simulink model "ASM_Traffic_MultiCore"  (R2026a)
settings: Solver=ode1  StartTime=SIM.tstart.v  StopTime=SIM.tend.v  FixedStep=SIM.StepSize.v
PostLoadFcn:
  | if any(exist('dsrtsu_mdlpostloadfcn', 'file') ~= 0), dsrtsu_mdlpostloadfcn('Execute', bdroot); end
  | try, asm_mdl_postloadfcn(bdroot, 'UpdateModel', 3600); catch, disp(lasterr); end,
InitFcn:
  | , if any(exist('rtifpga_mdlclblib', 'file') ~= 0), rtifpga_mdlclblib('Init', bdroot); end,
  | , if any(exist('dsmpb_private', 'file') ~= 0), dsmpb_private('dsmpb_mdlclblib', 'Init', bdroot); end,
model workspace (MAT data in the model file):
  asmReferencePath = [0 0.01 0.02 0.03 0.04 0.05 0.06 0.07 0.08 0.09 0.1 0.11 ... (350007 elements, 50001x7)]
  roadBounds : Simulink.Parameter (value not decoded)
  safetyAxes : Simulink.Parameter (value not decoded)
undefined symbols (not defined in the file): _to_, a0b2, ASM_BrakeHydraulics_DemoSystems, ASM_VehicleDynamics_DemoSystems, b98103fe8ad365046cd0, BrakeCircuit, controllerConfig, CPT, Crankshaft, DiscIntNeverNeededParam, dsmsi, FinalDriveAssembly, MDL, ModeSignals, mu, Pos_BrakePedal_Maneuver, rad, RefSignals, roadFamilyData, roadFamilyId, s_to_rpm, SIM, SoftECU, Suspension, Tire, Transmission
libraries: ASM_Traffic_lib x135, simulink x98, ASM_Utils_lib x77, ASM_VehicleDynamics_lib x70, ASM_Environment_lib x22, dsmpblib x20, dsmsilib x15, MDLD_Utils_lib x10, ASM_BrakeHydraulics_lib x3, sl_discontinuities x2
(part 27 of 65)

== system ASM_Traffic_MultiCore/Environment/Interface_Out/Plant_ModelSignals/Sw_TipShift_Maneuver[-1Down|0Off|1Up]_ ==
  In1 : Inport
  DummyGain : Gain  SaturateOnIntegerOverflow=on  OutDataTypeStr=Inherit: Same as input  ParamDataTypeStr=Inherit: Same as input
  Out1 : Outport  VectorParamsAs1DForOutWhenUnconnected=off
  wires:
  In1/1 -> DummyGain/1
  DummyGain/1 -> Out1/1

== system ASM_Traffic_MultiCore/Environment/Interface_Out/Plant_ModelSignals/Sw_Tire_Parameter_Set_CP[:][1|2|3|4]_ ==
  In1 : Inport
  Gain : Gain  SaturateOnIntegerOverflow=on  OutDataTypeStr=Inherit: Same as input  ParamDataTypeStr=Inherit: Same as input
  Out1 : Outport  VectorParamsAs1DForOutWhenUnconnected=off
  wires:
  In1/1 -> Gain/1
  Gain/1 -> Out1/1

== system ASM_Traffic_MultiCore/Environment/Interface_Out/Plant_ModelSignals/T_Ambient[degC]_ ==
  In1 : Inport
  Gain : Gain  SaturateOnIntegerOverflow=on  OutDataTypeStr=Inherit: Same as input  ParamDataTypeStr=Inherit: Same as input
  Out1 : Outport  VectorParamsAs1DForOutWhenUnconnected=off
  wires:
  In1/1 -> Gain/1
  Gain/1 -> Out1/1

== system ASM_Traffic_MultiCore/Environment/Interface_Out/Plant_ModelSignals/Trq_Driver_External[Nm]_ ==
  In1 : Inport
  Gain : Gain  SaturateOnIntegerOverflow=on  OutDataTypeStr=Inherit: Same as input  ParamDataTypeStr=Inherit: Same as input
  Out1 : Outport  VectorParamsAs1DForOutWhenUnconnected=off
  wires:
  In1/1 -> Gain/1
  Gain/1 -> Out1/1

== system ASM_Traffic_MultiCore/Environment/Interface_Out/Plant_ModelSignals/UnitVec_z_CP[:][x;y;z]_ ==
  In1 : Inport
  Gain : Gain  SaturateOnIntegerOverflow=on  OutDataTypeStr=Inherit: Same as input  ParamDataTypeStr=Inherit: Same as input
  Out1 : Outport  VectorParamsAs1DForOutWhenUnconnected=off
  wires:
  In1/1 -> Gain/1
  Gain/1 -> Out1/1

== system ASM_Traffic_MultiCore/Environment/Interface_Out/Plant_ModelSignals/Width_Deadzone_LatCtrl[m]_ ==
  In1 : Inport
  Gain : Gain  SaturateOnIntegerOverflow=on  OutDataTypeStr=Inherit: Same as input  ParamDataTypeStr=Inherit: Same as input
  Out1 : Outport  VectorParamsAs1DForOutWhenUnconnected=off
  wires:
  In1/1 -> Gain/1
  Gain/1 -> Out1/1

== system ASM_Traffic_MultiCore/Environment/Interface_Out/Plant_ModelSignals/Width_Fellows[m]_ ==
  In1 : Inport
  Gain : Gain  SaturateOnIntegerOverflow=on  OutDataTypeStr=Inherit: Same as input  ParamDataTypeStr=Inherit: Same as input
  Out1 : Outport  VectorParamsAs1DForOutWhenUnconnected=off
  wires:
  In1/1 -> Gain/1
  Gain/1 -> Out1/1

== system ASM_Traffic_MultiCore/Environment/Interface_Out/Plant_ModelSignals/a_x_Max[m|s2]_ ==
  In1 : Inport
  DummyGain : Gain  SaturateOnIntegerOverflow=on  OutDataTypeStr=Inherit: Same as input  ParamDataTypeStr=Inherit: Same as input
  Out1 : Outport  VectorParamsAs1DForOutWhenUnconnected=off
  wires:
  DummyGain/1 -> Out1/1
  In1/1 -> DummyGain/1

== system ASM_Traffic_MultiCore/Environment/Interface_Out/Plant_ModelSignals/a_x_Min[m|s2]_ ==
  In1 : Inport
  DummyGain : Gain  SaturateOnIntegerOverflow=on  OutDataTypeStr=Inherit: Same as input  ParamDataTypeStr=Inherit: Same as input
  Out1 : Outport  VectorParamsAs1DForOutWhenUnconnected=off
  wires:
  In1/1 -> DummyGain/1
  DummyGain/1 -> Out1/1

== system ASM_Traffic_MultiCore/Environment/Interface_Out/Plant_ModelSignals/a_x_Vehicle_Ref_TrafficDriver[m|s2]_ ==
  In1 : Inport
  Gain : Gain  SaturateOnIntegerOverflow=on  OutDataTypeStr=Inherit: Same as input  ParamDataTypeStr=Inherit: Same as input
  Out1 : Outport  VectorParamsAs1DForOutWhenUnconnected=off
  wires:
  Gain/1 -> Out1/1
  In1/1 -> Gain/1

== system ASM_Traffic_MultiCore/Environment/Interface_Out/Plant_ModelSignals/a_y_Max[m|s2]_ ==
  In1 : Inport
  DummyGain : Gain  SaturateOnIntegerOverflow=on  OutDataTypeStr=Inherit: Same as input  ParamDataTypeStr=Inherit: Same as input
  Out1 : Outport  VectorParamsAs1DForOutWhenUnconnected=off
  wires:
  DummyGain/1 -> Out1/1
  In1/1 -> DummyGain/1

== system ASM_Traffic_MultiCore/Environment/Interface_Out/Plant_ModelSignals/d_Total_Fellows[m]_ ==
  In1 : Inport
  Gain : Gain  SaturateOnIntegerOverflow=on  OutDataTypeStr=Inherit: Same as input  ParamDataTypeStr=Inherit: Same as input
  Out1 : Outport  VectorParamsAs1DForOutWhenUnconnected=off
  wires:
  In1/1 -> Gain/1
  Gain/1 -> Out1/1

== system ASM_Traffic_MultiCore/Environment/Interface_Out/Plant_ModelSignals/d_Vehicle_Road[m]_ ==
  In1 : Inport
  Gain : Gain  SaturateOnIntegerOverflow=on  OutDataTypeStr=Inherit: Same as input  ParamDataTypeStr=Inherit: Same as input
  Out1 : Outport  VectorParamsAs1DForOutWhenUnconnected=off
  wires:
  In1/1 -> Gain/1
  Gain/1 -> Out1/1

== system ASM_Traffic_MultiCore/Environment/Interface_Out/Plant_ModelSignals/n_Engine_Set[rpm]_ ==
  In1 : Inport
  DummyGain : Gain  SaturateOnIntegerOverflow=on  OutDataTypeStr=Inherit: Same as input  ParamDataTypeStr=Inherit: Same as input
  Out1 : Outport  VectorParamsAs1DForOutWhenUnconnected=off
  wires:
  In1/1 -> DummyGain/1
  DummyGain/1 -> Out1/1

== system ASM_Traffic_MultiCore/Environment/Interface_Out/Plant_ModelSignals/p_Ambient[Pa]_ ==
  In1 : Inport
  Gain : Gain  SaturateOnIntegerOverflow=on  OutDataTypeStr=Inherit: Same as input  ParamDataTypeStr=Inherit: Same as input
  Out1 : Outport  VectorParamsAs1DForOutWhenUnconnected=off
  wires:
  In1/1 -> Gain/1
  Gain/1 -> Out1/1

== system ASM_Traffic_MultiCore/Environment/Interface_Out/Plant_ModelSignals/q_dt_Vehicle_Init[6x1]_ ==
  In1 : Inport
  Gain : Gain  SaturateOnIntegerOverflow=on  OutDataTypeStr=Inherit: Same as input  ParamDataTypeStr=Inherit: Same as input
  Out1 : Outport  VectorParamsAs1DForOutWhenUnconnected=off
  wires:
  In1/1 -> Gain/1
  Gain/1 -> Out1/1

== system ASM_Traffic_MultiCore/Environment/Interface_Out/Plant_ModelSignals/s_Fellows_Ref[m]_ ==
  In1 : Inport
  Gain : Gain  SaturateOnIntegerOverflow=on  OutDataTypeStr=Inherit: Same as input  ParamDataTypeStr=Inherit: Same as input
  Out1 : Outport  VectorParamsAs1DForOutWhenUnconnected=off
  wires:
  In1/1 -> Gain/1
  Gain/1 -> Out1/1

== system ASM_Traffic_MultiCore/Environment/Interface_Out/Plant_ModelSignals/s_Total_Vehicle_Road[m]_ ==
  In1 : Inport
  Gain : Gain  SaturateOnIntegerOverflow=on  OutDataTypeStr=Inherit: Same as input  ParamDataTypeStr=Inherit: Same as input
  Out1 : Outport  VectorParamsAs1DForOutWhenUnconnected=off
  wires:
  Gain/1 -> Out1/1
  In1/1 -> Gain/1

== system ASM_Traffic_MultiCore/Environment/Interface_Out/Plant_ModelSignals/s_Vehicle_Init[m]_ ==
  In1 : Inport
  Gain : Gain  SaturateOnIntegerOverflow=on  OutDataTypeStr=Inherit: Same as input  ParamDataTypeStr=Inherit: Same as input
  Out1 : Outport  VectorParamsAs1DForOutWhenUnconnected=off
  wires:
  Gain/1 -> Out1/1
  In1/1 -> Gain/1

== system ASM_Traffic_MultiCore/Environment/Interface_Out/Plant_ModelSignals/s_Vehicle_Road[m]_ ==
  In1 : Inport
  Gain : Gain  SaturateOnIntegerOverflow=on  OutDataTypeStr=Inherit: Same as input  ParamDataTypeStr=Inherit: Same as input
  Out1 : Outport  VectorParamsAs1DForOutWhenUnconnected=off
  wires:
  In1/1 -> Gain/1
  Gain/1 -> Out1/1

== system ASM_Traffic_MultiCore/Environment/Interface_Out/Plant_ModelSignals/v_Rel_Fellows[m|s]_ ==
  In1 : Inport
  Gain : Gain  SaturateOnIntegerOverflow=on  OutDataTypeStr=Inherit: Same as input  ParamDataTypeStr=Inherit: Same as input
  Out1 : Outport  VectorParamsAs1DForOutWhenUnconnected=off
  wires:
  In1/1 -> Gain/1
  Gain/1 -> Out1/1

== system ASM_Traffic_MultiCore/Environment/Interface_Out/Plant_ModelSignals/v_Vehicle_Preview_Ref_Maneuver[m|s]_ ==
  In1 : Inport
  DummyGain : Gain  SaturateOnIntegerOverflow=on  OutDataTypeStr=Inherit: Same as input  ParamDataTypeStr=Inherit: Same as input
  Out1 : Outport  VectorParamsAs1DForOutWhenUnconnected=off
  wires:
  In1/1 -> DummyGain/1
  DummyGain/1 -> Out1/1

== system ASM_Traffic_MultiCore/Environment/Interface_Out/Plant_ModelSignals/v_Vehicle_Ref_Maneuver[km|h]_ ==
  In1 : Inport
  DummyGain : Gain  SaturateOnIntegerOverflow=on  OutDataTypeStr=Inherit: Same as input  ParamDataTypeStr=Inherit: Same as input
  Out1 : Outport  VectorParamsAs1DForOutWhenUnconnected=off
  wires:
  DummyGain/1 -> Out1/1
  In1/1 -> DummyGain/1

== system ASM_Traffic_MultiCore/Environment/Interface_Out/Plant_ModelSignals/v_Wind_Coor_Sys_E[x;y;z][m|s]_ ==
  In1 : Inport
  Gain : Gain  SaturateOnIntegerOverflow=on  OutDataTypeStr=Inherit: Same as input  ParamDataTypeStr=Inherit: Same as input
  Out1 : Outport  VectorParamsAs1DForOutWhenUnconnected=off
  wires:
  In1/1 -> Gain/1
  Gain/1 -> Out1/1

== system ASM_Traffic_MultiCore/Environment/Interface_Out/Plant_ModelSignals/x_Preview_DriverCurv[m]_ ==
  In1 : Inport
  Gain : Gain  SaturateOnIntegerOverflow=on  OutDataTypeStr=Inherit: Same as input  ParamDataTypeStr=Inherit: Same as input
  Out1 : Outport  VectorParamsAs1DForOutWhenUnconnected=off
  wires:
  In1/1 -> Gain/1
  Gain/1 -> Out1/1

== system ASM_Traffic_MultiCore/Environment/Interface_Out/Plant_ModelSignals/y_Preview_DriverCurv[m]_ ==
  In1 : Inport
  Gain : Gain  SaturateOnIntegerOverflow=on  OutDataTypeStr=Inherit: Same as input  ParamDataTypeStr=Inherit: Same as input
  Out1 : Outport  VectorParamsAs1DForOutWhenUnconnected=off
  wires:
  Gain/1 -> Out1/1
  In1/1 -> Gain/1

== system ASM_Traffic_MultiCore/Environment/Maneuver/PlantModel/ASMSignalCollector ==
  UserInterface : Inport
  VehicleInitStates : Inport  Port=2
  ModeSignals : Inport  Port=3
  RefSignals : Inport  Port=4
  Bus Creator : BusCreator  Inputs=7
  Bus Selector8 : BusSelector  OutputSignals=ManualControl.Testbench,ManualControl.ParkingBrake,ManualControl.StartButton,ManualControl.AutomaticTransmission.Sw_TipShift[-1Down|0Off|1Up]
  Replace_ModeSignals : BusAssignment  AssignedSignals=ModeSignals,RefSignals
  Maneuver_Signals : Outport  VectorParamsAs1DForOutWhenUnconnected=off
  wires:
  VehicleInitStates/1 -> Bus Creator/3
  Bus Selector8/1 -> Bus Creator/4  "<Testbench>"
  Bus Creator/1 -> Maneuver_Signals/1  "Maneuver"
  [ASMBUS_Environment_Mnvr_UserSignalsCustomized] -> Bus Creator/2
  [ASMBUS_Environment_ManeuverScheduler] -> Replace_ModeSignals/1
  Bus Selector8/2 -> Bus Creator/5  "<ParkingBrake>"
  Bus Selector8/3 -> Bus Creator/6  "<StartButton>"
  Bus Selector8/4 -> Bus Creator/7  "<Sw_TipShift[-1Down|0Off|1Up]>"
  ModeSignals/1 -> Replace_ModeSignals/2
  RefSignals/1 -> Replace_ModeSignals/3
  Replace_ModeSignals/1 -> Bus Creator/1  "ManeuverScheduler"
  UserInterface/1 -> Bus Selector8/1

== system ASM_Traffic_MultiCore/Environment/Maneuver/PlantModel/Customize_UserSignals ==
  UserSignals_In : Inport
  Bus Creator : BusCreator  Inputs=14
  Bus Selector1 : BusSelector  OutputSignals=User1[],User2[],User3[],User4[],User5[],User6[],User7[],User8[],User9[],User10[],User11[],User12[],User13[],User14[]
  CustomizedUserSignals : Subsystem
  ASMSignalBus : Outport  VectorParamsAs1DForOutWhenUnconnected=off
  UserSignals_Customized : Outport  Port=2  VectorParamsAs1DForOutWhenUnconnected=off
  wires:
  CustomizedUserSignals/8(Mnv_DataStream_8[]) -> Bus Creator/8
  CustomizedUserSignals/7(Mnv_DataStream_7[]) -> Bus Creator/7
  CustomizedUserSignals/6(Mnv_DataStream_6[]) -> Bus Creator/6
  CustomizedUserSignals/5(Mnv_DataStream_5[]) -> Bus Creator/5
  Bus Selector1/8 -> CustomizedUserSignals/8(User8[])  "<User8[]>"
  Bus Selector1/7 -> CustomizedUserSignals/7(User7[])  "<User7[]>"
  Bus Selector1/6 -> CustomizedUserSignals/6(User6[])  "<User6[]>"
  Bus Selector1/5 -> CustomizedUserSignals/5(User5[])  "<User5[]>"
  Bus Selector1/4 -> CustomizedUserSignals/4(User4[])  "<User4[]>"
  Bus Selector1/3 -> CustomizedUserSignals/3(User3[])  "<User3[]>"
  CustomizedUserSignals/3(ASM_Vehicle_TurnLights[]) -> Bus Creator/3
  CustomizedUserSignals/4(ECU_Commands[]) -> Bus Creator/4
  UserSignals_In/1 -> Bus Selector1/1
  Bus Creator/1 -> ASMSignalBus/1, UserSignals_Customized/1  "UserSignals_Customized"
  Bus Selector1/1 -> CustomizedUserSignals/1(User1[])  "<User1[]>"
  Bus Selector1/2 -> CustomizedUserSignals/2(User2[])  "<User2[]>"
  CustomizedUserSignals/1(ExternalSegmentEnd_Mode[]) -> Bus Creator/1
  CustomizedUserSignals/2(ExternalSegmentEnd_Value[]) -> Bus Creator/2
  Bus Selector1/9 -> CustomizedUserSignals/9(User9[])  "<User9[]>"
  Bus Selector1/10 -> CustomizedUserSignals/10(User10[])  "<User10[]>"
  Bus Selector1/11 -> CustomizedUserSignals/11(User11[])  "<User11[]>"
  Bus Selector1/12 -> CustomizedUserSignals/12(User12[])  "<User12[]>"
  Bus Selector1/13 -> CustomizedUserSignals/13(User13[])  "<User13[]>"
  Bus Selector1/14 -> CustomizedUserSignals/14(User14[])  "<User14[]>"
  CustomizedUserSignals/9(Mnv_DoorFL[]) -> Bus Creator/9
  CustomizedUserSignals/10(Mnv_DoorFR[]) -> Bus Creator/10
  CustomizedUserSignals/11(Mnv_DoorRL[]) -> Bus Creator/11
  CustomizedUserSignals/12(Mnv_DoorRR[]) -> Bus Creator/12
  CustomizedUserSignals/13(Mnv_Hood[]) -> Bus Creator/13
  CustomizedUserSignals/14(Mnv_Trunk[]) -> Bus Creator/14

== system ASM_Traffic_MultiCore/Environment/Maneuver/PlantModel/ExternalSegmentEnd ==
  In : Inport
  UserSignals_Customized : Inport  Port=2
  AvoidAlgLoop{1..9} (9 alike) : UnitDelay  SampleTime=-1
  Bus Selector : BusSelector  OutputSignals=ExternalSegmentEnd_Mode[],ExternalSegmentEnd_Value[]
  Bus Selector1 : BusSelector  OutputSignals=Plant.Traffic_Signals_toEnvironment.UserSignals_Customized.ManeuverSegmentEndTrigger[0|1]
  Bus Selector2 : BusSelector  OutputSignals=Plant.Road_ASMVeh.s_Veh_Road[m]
  Bus Selector3 : BusSelector  OutputSignals=Road,Interface_In,Sensors,Traffic
  Bus Selector4 : BusSelector  OutputSignals=ExternalModel.RollRate_Vehicle_CoG[deg|s]
  Bus Selector5 : BusSelector  OutputSignals=Plant.Object_Sensor_3D.Sensor_1_Front_Long,Plant.Object_Sensor_3D.Sensor_3_Rear
  Bus Selector6 : BusSelector  OutputSignals=ExternalModel.AEB[0|1],ExternalModel.FCW[0|1]
  Bus Selector7 : BusSelector  OutputSignals=SensorOutput.Dist_Object[m]
  Bus Selector8 : BusSelector  OutputSignals=SensorOutput.Dist_Object[m]
  Const_External_SegmentEnd_10[0|1] : Constant  Value=0
  Const_External_SegmentEnd_11_25 : Constant  Value=zeros(15,1)
  Const_External_SegmentEnd_5[0|1] : Constant  Value=0
  Const_External_SegmentEnd_6[0|1] : Constant  Value=0
  Const_External_SegmentEnd_7[0|1] : Constant  Value=0
  Const_External_SegmentEnd_8[0|1] : Constant  Value=0
  Const_External_SegmentEnd_9[0|1] : Constant  Value=0
  Dist_Front_Min : Subsystem
  Dist_Rear_Min : Subsystem
  Mux : Mux  Inputs=[1 1 1 1 1 1 1 1 1 1 15]
  SegmentEndTrigger : Subsystem
  External_SegmentEnd[0|1] : Outport  VectorParamsAs1DForOutWhenUnconnected=off
  wires:
  Bus Selector7/1 -> Dist_Front_Min/1(Dist_Front[m])  "<Dist_Object[m]>"
  AvoidAlgLoop9/1 -> Mux/4
  AvoidAlgLoop8/1 -> Mux/3
  Bus Selector6/2 -> AvoidAlgLoop9/1  "<FCW[0|1]>"
  Bus Selector6/1 -> AvoidAlgLoop8/1  "<AEB[0|1]>"
  Const_External_SegmentEnd_5[0|1]/1 -> Mux/5
  Const_External_SegmentEnd_6[0|1]/1 -> Mux/6
  Const_External_SegmentEnd_7[0|1]/1 -> Mux/7
  Const_External_SegmentEnd_8[0|1]/1 -> Mux/8
  Const_External_SegmentEnd_9[0|1]/1 -> Mux/9
  Const_External_SegmentEnd_10[0|1]/1 -> Mux/10
  Mux/1 -> External_SegmentEnd[0|1]/1
  Bus Selector3/4 -> Bus Selector1/1  "<Traffic>"
  Bus Selector1/1 -> AvoidAlgLoop6/1  "<ManeuverSegmentEndTrigger[0|1]>"
  AvoidAlgLoop6/1 -> Mux/2
  UserSignals_Customized/1 -> Bus Selector/1
  Bus Selector/1 -> AvoidAlgLoop1/1  "<ExternalSegmentEnd_Mode[]>"
  Bus Selector/2 -> AvoidAlgLoop2/1  "<ExternalSegmentEnd_Value[]>"
  Bus Selector3/2 -> Bus Selector6/1, Bus Selector4/1  "<Interface_In>"
  Bus Selector4/1 -> AvoidAlgLoop4/1  "<RollRate_Vehicle_CoG[deg|s]>"
  Bus Selector2/1 -> AvoidAlgLoop3/1  "<s_Veh_Road[m]>"
  AvoidAlgLoop1/1 -> SegmentEndTrigger/1(ExternalSegmentEnd_Mode[])
  AvoidAlgLoop2/1 -> SegmentEndTrigger/2(ExternalSegmentEnd_Value[])
  AvoidAlgLoop3/1 -> SegmentEndTrigger/3(s_Road[m])
  AvoidAlgLoop4/1 -> SegmentEndTrigger/4(RollRate_Vehicle[deg|s])
  Dist_Front_Min/1(Out1) -> AvoidAlgLoop5/1
  Dist_Rear_Min/1(Out1) -> AvoidAlgLoop7/1
  AvoidAlgLoop7/1 -> SegmentEndTrigger/6(Distance_Rear[m])
  AvoidAlgLoop5/1 -> SegmentEndTrigger/5(Distance_Front[m])
  SegmentEndTrigger/1(External_SegmentEnd[0|1]) -> Mux/1
  Const_External_SegmentEnd_11_25/1 -> Mux/11
  In/1 -> Bus Selector3/1
  Bus Selector3/1 -> Bus Selector2/1  "<Road>"
  Bus Selector3/3 -> Bus Selector5/1  "<Sensors>"
  Bus Selector5/1 -> Bus Selector7/1  "<Sensor_1_Front_Long>"
  Bus Selector5/2 -> Bus Selector8/1  "<Sensor_3_Rear>"
  Bus Selector8/1 -> Dist_Rear_Min/1(Dist_Rear[m])  "<Dist_Object[m]>"

== system ASM_Traffic_MultiCore/Environment/Maneuver/PlantModel/ExternalUserData ==
  Angle_SteeringWheel[deg] : Constant  Value=0
  Bus Creator2 : BusCreator  Inputs=10
  Gear[] : Constant  Value=0
  LaneIdx_Ref[] : Constant  Value=0
  Pos_AccPedal[%] : Constant  Value=0
  Pos_BrakePedal[%] : Constant  Value=0
  Pos_ClutchPedal[%] : Constant  Value=100
  "SelectorLever[] " : Constant  Value=0
  Trq_Steering[Nm] : Constant  Value=0
  d_Ref[m] : Constant  Value=0
  v_Vehicle_Ref[m|s] : Constant  Value=0
  External_ReferenceSignals : Outport  VectorParamsAs1DForOutWhenUnconnected=off
  wires:
  "SelectorLever[] "/1 -> Bus Creator2/10  "SelectorLever[]"
  Trq_Steering[Nm]/1 -> Bus Creator2/9  "Trq_Steering[Nm]"
  Angle_SteeringWheel[deg]/1 -> Bus Creator2/5  "Angle_SteeringWheel[deg]"
  Gear[]/1 -> Bus Creator2/4  "Gear[]"
  Pos_ClutchPedal[%]/1 -> Bus Creator2/3  "Pos_ClutchPedal[%]"
  Pos_BrakePedal[%]/1 -> Bus Creator2/2  "Pos_BrakePedal[%]"
  Pos_AccPedal[%]/1 -> Bus Creator2/1  "Pos_AccPedal[%]"
  v_Vehicle_Ref[m|s]/1 -> Bus Creator2/6  "v_Vehicle_Ref[m|s]"
  d_Ref[m]/1 -> Bus Creator2/7  "d_Ref[m]"
  LaneIdx_Ref[]/1 -> Bus Creator2/8  "LaneIdx_Ref[]"
  Bus Creator2/1 -> External_ReferenceSignals/1

== system ASM_Traffic_MultiCore/Environment/Maneuver/PlantModel/InitialVehicleStates ==
  note: Set v_x_Init to zero if Keep_VehiclePosition is enabled or the maneuver state is BRAKE or WAIT.
  note: Use v_x_Init from VehicleInitStates_External if the maneuver state is INIT_MANUAL or MANUAL; else use v_x_Init from the maneuver scheduler.
  UserInterface : Inport
  MdlControl : Inport  Port=2
  InitialVehStates : Inport  Port=3
  Info[] : Inport  Port=4
  Bus Creator1 : BusCreator  Inputs=2
  Bus Selector10 : BusSelector  OutputSignals=Vehicle_Init
  Bus Selector2 : BusSelector  OutputSignals=v_Vehicle_Init[km|h]
  Bus Selector3 : BusSelector  OutputSignals=Keep_VehiclePosition[0|1]
  Bus Selector4 : BusSelector  OutputSignals=Reset_VehicleStates[0|1]
  Bus Selector5 : BusSelector  OutputSignals=ManeuverState[],CurrentSequence[],CurrentSegment[]
  Bus to Vector : BusToVector
  Const_zero_v_x_Init[km|h] : Constant  Value=0  VectorParams1D=off
  DRIVETRAIN_INIT : ASM_Environment_lib/Environment/Maneuver/DRIVETRAIN_INIT  StepSize=SIM.StepSize  ASMProperties=struct('Name','DRIVETRAIN_INIT','Version','1.0','Library','ASM_Environment_lib')  ASMInstanceName=drivetrain_init  ASMInstanceID=1
  Demux : Demux  Outputs=[1 1 1 3]
  Keep_VehiclePosition_enabled : simulink/Logic and Bit Operations/Compare To Constant  relop===  const=1  OutDataTypeStr=uint8  ZeroCross=off
  Mux : Mux  Inputs=3
  Mux1 : Mux  Inputs=[3 3]
  OR : Logic  Operator=OR  Inputs=3  IconShape=distinctive  AllPortsSameDT=off  OutDataTypeStr=boolean
  OR1 : Logic  Operator=OR  IconShape=distinctive  AllPortsSameDT=off  OutDataTypeStr=boolean
  State_BRAKE : simulink/Logic and Bit Operations/Compare To Constant  relop===  const=4  OutDataTypeStr=uint8  ZeroCross=off
  State_INIT_MANUAL : simulink/Logic and Bit Operations/Compare To Constant  relop===  const=6  OutDataTypeStr=uint8  ZeroCross=off
  State_MANUAL : simulink/Logic and Bit Operations/Compare To Constant  relop===  const=7  OutDataTypeStr=uint8  ZeroCross=off
  State_WAIT : simulink/Logic and Bit Operations/Compare To Constant  relop===  const=5  OutDataTypeStr=uint8  ZeroCross=off
  Sw_KeepVehiclePosition_Dependency : Gain
  Sw_ManeuverState_Dependency : Gain
  Switch : Switch  Criteria=u2 ~= 0  SaturateOnIntegerOverflow=off  InputSameDT=off
  Switch1 : Switch  Criteria=u2 ~= 0  SaturateOnIntegerOverflow=off  InputSameDT=off
  Unit Delay : UnitDelay  SampleTime=-1
  UnitConversion : ASM_Utils_lib/UnitConversion/UnitConversion  Selection=km/h_to_m/s
  VehicleInitStates : Outport  VectorParamsAs1DForOutWhenUnconnected=off
  Flag_Init_Drivetrain[0InProgress|1Finished] : Outport  Port=2  VectorParamsAs1DForOutWhenUnconnected=off
  wires:
  Demux/3 -> Mux/3  "vz"
  Demux/2 -> Mux/2  "vy"
  Bus Creator1/1 -> VehicleInitStates/1  "VehicleInitStates"
  Mux/1 -> UnitConversion/1
  Demux/4 -> Mux1/2  "w_Init[x;y;z][rad|s]"
  Unit Delay/1 -> Mux/1  "vx"
  Mux1/1 -> Bus Creator1/1  "q_dt_Vehicle_Init[6x1]"
  Demux/1 -> Switch1/1
  State_BRAKE/1 -> OR/2
  State_WAIT/1 -> OR/3
  Sw_ManeuverState_Dependency/1 -> State_BRAKE/1, State_MANUAL/1, State_INIT_MANUAL/1, State_WAIT/1
  Sw_KeepVehiclePosition_Dependency/1 -> Keep_VehiclePosition_enabled/1
  Keep_VehiclePosition_enabled/1 -> OR/1
  OR/1 -> Switch/2
  Switch1/1 -> Switch/3
  Switch/1 -> Unit Delay/1
  State_INIT_MANUAL/1 -> OR1/1
  State_MANUAL/1 -> OR1/2
  OR1/1 -> Switch1/2
  Bus to Vector/1 -> Demux/1
  UnitConversion/1 -> Mux1/1  "v_Init[x;y;z][m|s]"
  Bus Selector10/1 -> Bus to Vector/1  "<Vehicle_Init>"
  UserInterface/1 -> Bus Selector10/1
  Bus Selector3/1 -> Sw_KeepVehiclePosition_Dependency/1  "<Keep_VehiclePosition[0|1]>"
  MdlControl/1 -> Bus Selector4/1, Bus Selector3/1
  Bus Selector2/1 -> DRIVETRAIN_INIT/1, Switch1/3  "<v_Vehicle_Init[km|h]>"
  InitialVehStates/1 -> Bus Selector2/1
  Const_zero_v_x_Init[km|h]/1 -> Switch/1
  Bus Selector5/3 -> DRIVETRAIN_INIT/4  "<CurrentSegment[]>"
  Bus Selector5/1 -> Sw_ManeuverState_Dependency/1, DRIVETRAIN_INIT/2  "<ManeuverState[]>"
  Bus Selector5/2 -> DRIVETRAIN_INIT/3  "<CurrentSequence[]>"
  Info[]/1 -> Bus Selector5/1
  Bus Selector4/1 -> DRIVETRAIN_INIT/5  "<Reset_VehicleStates[0|1]>"
  DRIVETRAIN_INIT/1 -> Bus Creator1/2  "Enable_v_Init[0|1]"
  DRIVETRAIN_INIT/2 -> Flag_Init_Drivetrain[0InProgress|1Finished]/1

== system ASM_Traffic_MultiCore/Environment/Maneuver/PlantModel/LastValues ==
  In : Inport
  Maneuver_RefSignals : Inport  Port=2
  AvoidAlgLoop_AccPed : UnitDelay  SampleTime=-1
  AvoidAlgLoop_BrakePed : UnitDelay  SampleTime=-1
  AvoidAlgLoop_ClutchPed : UnitDelay  SampleTime=-1
  AvoidAlgLoop_Gear : UnitDelay  SampleTime=-1
  AvoidAlgLoop_Steer{,1..4} (5 alike) : UnitDelay  SampleTime=-1
  Bus Creator3 : BusCreator  Inputs=9
  Bus Selector1 : BusSelector  OutputSignals=ExternalModel.Angle_SteeringWheel_SteeringSystem[deg],ExternalModel.Trq_SteeringWheel_SteeringSystem[Nm]
  Bus Selector2 : BusSelector  OutputSignals=ExternalModel.Pos_AccPedal[%],ExternalModel.Pos_BrakePedal[%],ExternalModel.Pos_ClutchPedal[%],ExternalModel.Gear[],ExternalModel.SelectorLever[-3T|-2P|-1R|0N|1D],ExternalModel.Angle_SteeringWheel[deg]
  Bus Selector3 : BusSelector  OutputSignals=Sw_SteeringMode_Maneuver[1Angle|2Trq]
  Bus Selector4 : BusSelector  OutputSignals=Interface_In,Road
  Bus Selector5 : BusSelector  OutputSignals=Plant.Road_ASMVeh.d_Total_Veh_Road[m],Plant.Road_ASMVeh.LaneIdx_Total_Veh_Road[]
  Multiport Switch : MultiPortSwitch  Inputs=2  SaturateOnIntegerOverflow=off  InputSameDT=off
  LastValues : Outport  VectorParamsAs1DForOutWhenUnconnected=off
  wires:
  Bus Selector5/1 -> AvoidAlgLoop_Steer1/1  "<d_Total_Veh_Road[m]>"
  Bus Selector5/2 -> AvoidAlgLoop_Steer2/1  "<LaneIdx_Total_Veh_Road[]>"
  Bus Creator3/1 -> LastValues/1
  AvoidAlgLoop_Steer2/1 -> Bus Creator3/7  "LaneIdx_Total_Veh_Road_Last[]"
  AvoidAlgLoop_Steer1/1 -> Bus Creator3/6  "d_Total_Veh_Road_Last[m]"
  AvoidAlgLoop_Steer/1 -> Bus Creator3/5  "Angle_SteeringWheel_Last[deg]"
  AvoidAlgLoop_Gear/1 -> Bus Creator3/4  "Gear_Last[]"
  AvoidAlgLoop_ClutchPed/1 -> Bus Creator3/3  "Pos_ClutchPedal_Last[%]"
  AvoidAlgLoop_BrakePed/1 -> Bus Creator3/2  "Pos_BrakePedal_Last[%]"
  AvoidAlgLoop_AccPed/1 -> Bus Creator3/1  "Pos_AccPedal_Last[%]"
  Bus Selector2/1 -> AvoidAlgLoop_AccPed/1  "<Pos_AccPedal[%]>"
  Bus Selector2/2 -> AvoidAlgLoop_BrakePed/1  "<Pos_BrakePedal[%]>"
  Bus Selector2/3 -> AvoidAlgLoop_ClutchPed/1  "<Pos_ClutchPedal[%]>"
  Bus Selector2/4 -> AvoidAlgLoop_Gear/1  "<Gear[]>"
  AvoidAlgLoop_Steer3/1 -> Bus Creator3/8  "Trq_SteeringWheel_Last[Nm]"
  Bus Selector1/2 -> AvoidAlgLoop_Steer3/1  "<Trq_SteeringWheel_SteeringSystem[Nm]>"
  Bus Selector2/6 -> Multiport Switch/2  "<Angle_SteeringWheel[deg]>"
  Maneuver_RefSignals/1 -> Bus Selector3/1
  Bus Selector3/1 -> Multiport Switch/1  "<Sw_SteeringMode_Maneuver[1Angle|2Trq]>"
  Multiport Switch/1 -> AvoidAlgLoop_Steer/1
  Bus Selector1/1 -> Multiport Switch/3  "<Angle_SteeringWheel_SteeringSystem[deg]>"
  AvoidAlgLoop_Steer4/1 -> Bus Creator3/9  "SelectorLever_Last[]"
  Bus Selector2/5 -> AvoidAlgLoop_Steer4/1  "<SelectorLever[-3T|-2P|-1R|0N|1D]>"
  In/1 -> Bus Selector4/1
  Bus Selector4/2 -> Bus Selector5/1  "<Road>"
  Bus Selector4/1 -> Bus Selector1/1, Bus Selector2/1  "<Interface_In>"

== system ASM_Traffic_MultiCore/Environment/Maneuver/PlantModel/ManeuverReset ==
  UserInterface : Inport
  In : Inport  Port=2
  Bus Selector1 : BusSelector  OutputSignals=ExternalModel.Mode_Transmission[1Manual|2Automatic]
  Bus Selector12 : BusSelector  OutputSignals=ExternalModel.Mode_Drivetrain[1|2|3|4|5]
  Bus Selector2 : BusSelector  OutputSignals=Sw_ManeuverControl.Reset[0|1]
  Bus Selector3 : BusSelector  OutputSignals=Interface_In
  Constant : Constant
  DTC : DataTypeConversion
  DetectChange : simulink/Logic and Bit Operations/Detect Change  vinit=0  OutDataTypeStr=boolean
  DetectChange1 : simulink/Logic and Bit Operations/Detect Change  vinit=0  OutDataTypeStr=boolean
  IgnoreSimStart : Product  SaturateOnIntegerOverflow=on  OutDataTypeStr=Inherit: Same as first input
  LogOp_Or_ExtReset : Logic  Operator=OR  IconShape=distinctive  AllPortsSameDT=off
  Memory : Memory
  OR : Logic  Operator=OR  IconShape=distinctive  AllPortsSameDT=off  OutDataTypeStr=boolean
  Reset_IfModeSwitched : Gain  SaturateOnIntegerOverflow=on  OutDataTypeStr=Inherit: Same as input  ParamDataTypeStr=Inherit: Same as input
  Sat_DrvTrnMode : Saturate  UpperLimit=5  LowerLimit=1
  Sat_TrmMode : Saturate  UpperLimit=2  LowerLimit=1
  Reset[0|1] : Outport  VectorParamsAs1DForOutWhenUnconnected=off
  wires:
  Sat_DrvTrnMode/1 -> DetectChange/1
  IgnoreSimStart/1 -> Reset_IfModeSwitched/1
  Sat_TrmMode/1 -> DetectChange1/1
  OR/1 -> DTC/1
  Bus Selector12/1 -> Sat_DrvTrnMode/1  "<Mode_Drivetrain[1|2|3|4|5]>"
  Bus Selector1/1 -> Sat_TrmMode/1  "<Mode_Transmission[1Manual|2Automatic]>"
  DetectChange/1 -> OR/1
  DetectChange1/1 -> OR/2
  Memory/1 -> IgnoreSimStart/2
  Constant/1 -> Memory/1
  DTC/1 -> IgnoreSimStart/1
  Bus Selector2/1 -> LogOp_Or_ExtReset/1  "<Reset[0|1]>"
  UserInterface/1 -> Bus Selector2/1
  Reset_IfModeSwitched/1 -> LogOp_Or_ExtReset/2
  LogOp_Or_ExtReset/1 -> Reset[0|1]/1
  In/1 -> Bus Selector3/1
  Bus Selector3/1 -> Bus Selector1/1, Bus Selector12/1  "<Interface_In>"

== system ASM_Traffic_MultiCore/Environment/Maneuver/PlantModel/ReplaceBrake ==
  In : Inport
  RefSignals_In : Inport  Port=2
  Info[] : Inport  Port=3
  AND : Logic  IconShape=distinctive  AllPortsSameDT=off  OutDataTypeStr=boolean
  Bus Assignment : BusAssignment  AssignedSignals=Pos_BrakePedal_Maneuver[%]
  Bus Selector : BusSelector  OutputSignals=Pos_BrakePedal_Maneuver[%]
  Bus Selector1 : BusSelector  OutputSignals=Interface_In
  Bus Selector12 : BusSelector  OutputSignals=ExternalModel.Sw_MasterBrakeCylinder_Mode[1linear|2physical|3Booster]
  Bus Selector5 : BusSelector  OutputSignals=ManeuverState[]
  Const_Replace_Pos_BrakePedal[%] : Constant  Value=65
  OR : Logic  Operator=OR  IconShape=distinctive  AllPortsSameDT=off  OutDataTypeStr=boolean
  State_Brake : simulink/Logic and Bit Operations/Compare To Constant  relop===  const=4  OutDataTypeStr=boolean
  State_Wait : simulink/Logic and Bit Operations/Compare To Constant  relop===  const=5  OutDataTypeStr=boolean
  Switch : Switch  Criteria=u2 ~= 0  SaturateOnIntegerOverflow=off  InputSameDT=off
  Type_Physical : simulink/Logic and Bit Operations/Compare To Constant  relop===  const=2  OutDataTypeStr=boolean
  RefSignals : Outport  VectorParamsAs1DForOutWhenUnconnected=off
  wires:
  Bus Selector5/1 -> State_Wait/1, State_Brake/1  "<ManeuverState[]>"
  Bus Selector/1 -> Switch/3  "<Pos_BrakePedal_Maneuver[%]>"
  RefSignals_In/1 -> Bus Selector/1, Bus Assignment/1
  Bus Assignment/1 -> RefSignals/1  "RefSignals"
  Bus Selector12/1 -> Type_Physical/1  "<Sw_MasterBrakeCylinder_Mode[1linear|2physical|3Booster]>"
  State_Brake/1 -> OR/1
  State_Wait/1 -> OR/2
  OR/1 -> AND/2
  Type_Physical/1 -> AND/1
  AND/1 -> Switch/2
  Const_Replace_Pos_BrakePedal[%]/1 -> Switch/1
  Switch/1 -> Bus Assignment/2
  In/1 -> Bus Selector1/1
  Info[]/1 -> Bus Selector5/1
  Bus Selector1/1 -> Bus Selector12/1  "<Interface_In>"

== system ASM_Traffic_MultiCore/Environment/Maneuver/PlantModel/ReplaceSelectorLever_Mode ==
  UserInterface : Inport
  ModeSignals_In : Inport  Port=2
  Bus Assignment : BusAssignment  AssignedSignals=Mode_SelectorLever[1Stim|2Driver]
  Bus Selector : BusSelector  OutputSignals=Mode_SelectorLever[1Stim|2Driver]
  Bus Selector8 : BusSelector  OutputSignals=Sw_ManeuverControl.Sw_ManualDriving[1ManSched|2Manual],ManualControl.AutomaticTransmission.Mode_SelectorLever[1Stim|2Driver]
  Bus to Vector : BusToVector
  Multiport Switch : MultiPortSwitch  Inputs=2  DiagnosticForDefault=Warning  SaturateOnIntegerOverflow=off  InputSameDT=off
  ModeSignals : Outport  VectorParamsAs1DForOutWhenUnconnected=off
  wires:
  ModeSignals_In/1 -> Bus Selector/1, Bus Assignment/1
  Bus to Vector/1 -> Multiport Switch/1
  Bus Selector/1 -> Multiport Switch/2  "<Mode_SelectorLever[1Stim|2Driver]>"
  Multiport Switch/1 -> Bus Assignment/2
  Bus Assignment/1 -> ModeSignals/1  "ModeSignals"
  Bus Selector8/1 -> Bus to Vector/1  "<Sw_ManualDriving[1ManSched|2Manual]>"
  UserInterface/1 -> Bus Selector8/1
  Bus Selector8/2 -> Multiport Switch/3  "<Mode_SelectorLever[1Stim|2Driver]>"

== system ASM_Traffic_MultiCore/Environment/Maneuver/PlantModel/SimulationControl ==
  UserInterface : Inport
  In : Inport  Port=2
  Abs : Abs  SaturateOnIntegerOverflow=off
  Bus Selector1 : BusSelector  OutputSignals=SimulationControl.MaxAngleRollPitch.Max_Angle_Roll[deg],SimulationControl.MaxAngleRollPitch.Max_Angle_Pitch[deg],SimulationControl.Sw_Keep_VehiclePosition[0Off|1On]
  Bus Selector2 : BusSelector  OutputSignals=Interface_In
  Bus Selector4 : BusSelector  OutputSignals=ExternalModel.Angle_Vehicle_CoorSys_E[x;y;z][deg]
  Demux : Demux  Outputs=3
  Logical Operator : Logic  Operator=OR  Inputs=1  IconShape=distinctive  AllPortsSameDT=off  OutDataTypeStr=boolean
  Logical Operator1 : Logic  IconShape=distinctive  AllPortsSameDT=off
  Memory : UnitDelay  SampleTime=-1
  Mux : Mux  Inputs=2
  Mux1 : Mux  Inputs=2
  Relational Operator : RelationalOperator  Operator=>  OutDataTypeStr=boolean  InputSameDT=off
  Terminator17 : Terminator
  Keep_VehiclePosition[0|1] : Outport  VectorParamsAs1DForOutWhenUnconnected=off
  wires:
  Bus Selector1/2 -> Mux/2  "<Max_Angle_Pitch[deg]>"
  Bus Selector1/1 -> Mux/1  "<Max_Angle_Roll[deg]>"
  Bus Selector1/3 -> Logical Operator1/2  "<Sw_Keep_VehiclePosition[0Off|1On]>"
  UserInterface/1 -> Bus Selector1/1
  Relational Operator/1 -> Logical Operator/1
  Abs/1 -> Relational Operator/1
  Logical Operator/1 -> Memory/1
  Mux/1 -> Relational Operator/2
  Mux1/1 -> Abs/1
  Memory/1 -> Logical Operator1/1
  Logical Operator1/1 -> Keep_VehiclePosition[0|1]/1
  In/1 -> Bus Selector2/1
  Bus Selector2/1 -> Bus Selector4/1  "<Interface_In>"
  Demux/3 -> Terminator17/1
  Bus Selector4/1 -> Demux/1  "<Angle_Vehicle_CoorSys_E[x;y;z][deg]>"
  Demux/1 -> Mux1/1
  Demux/2 -> Mux1/2

== system ASM_Traffic_MultiCore/Environment/Maneuver/UserInterface/ASMSignalBus_Plant ==
  In : Inport
  Terminator : Terminator
  tag scope: ASMBUS_Environment_Maneuver=global
  wires:
  [ASMBUS_Environment_Maneuver] -> Terminator/1
  In/1 -> [ASMBUS_Environment_Maneuver]

== system ASM_Traffic_MultiCore/Environment/Maneuver/UserInterface/DISP_Plant ==
  In : Inport
  ASM_Vehicle_TurnLights[] : Subsystem
      mask Display: disp('')
  Angle_SteeringWheel_Maneuver[deg] : Subsystem
      mask Display: disp('')
  Bus Selector : BusSelector  OutputSignals=ManeuverScheduler.Info,ManeuverScheduler.MdlControl,ManeuverScheduler.ModeSignals,ManeuverScheduler.RefSignals,UserSignals_Customized
  Bus Selector1 : BusSelector  OutputSignals=CurrentSegment[],CurrentSequence[],t_local[s],s_local[m],ManeuverTime[s],ManeuverState[]
  Bus Selector2 : BusSelector  OutputSignals=Reset_VehicleStates[0|1],RoadControl[]
  Bus Selector3 : BusSelector  OutputSignals=Mode_AccBr[1Stim|2Driver],Mode_GearClutch[1Stim|2Driver|3OpenClutch|4RefGear],LatDriver[1LatCtrl1|2LatCtrl2],Mode_LatCtrl[1Pos|2Yaw],Mode_AdaptVelocityToRoad[1Off|2On],Mode_SelectorLever[1Stim|2Driver],Mode_TrafficDriver[1Off|2On],Mode_RelativeLane[0CenterLane|1PreferredLane]
  Bus Selector4 : BusSelector  OutputSignals=Pos_AccPedal_Maneuver[%],Pos_BrakePedal_Maneuver[%],Pos_ClutchPedal_Maneuver[%],Angle_SteeringWheel_Maneuver[deg],Gear_Maneuver[],SelectorLever_Maneuver[],d_Maneuver[m],LaneIdx_Maneuver[],v_Vehicle_Ref_Maneuver[m|s],v_Vehicle_Ref_Maneuver[km|h],v_Vehicle_Ref_Preview_Maneuver[m|s],v_Vehicle_Ref_Preview_State[0Invalid|1CurrentSeg|2NextSeg]
  Bus Selector5 : BusSelector  OutputSignals=ASM_Vehicle_TurnLights[]
  CurrentSegment[] : Subsystem
      mask Display: disp('')
  CurrentSequence[] : Subsystem
      mask Display: disp('')
  Driver : Scope  NumInputPorts=6
      settings: TimeSpan=5  DataLoggingMaxPoints=20000  DataLoggingDecimation=10  DataLoggingVariableName=ScopeData5
  Gear_Maneuver[] : Subsystem
      mask Display: disp('')
  LaneIdx_Maneuver[] : Subsystem
      mask Display: disp('')
  LatDriver[1LatCtrl|2LatCtrl2] : Subsystem
      mask Display: disp('')
  LateralOffset : Scope  NumInputPorts=2
      settings: TimeSpan=5  DataLoggingMaxPoints=20000  DataLoggingDecimation=10  DataLoggingVariableName=ScopeData4
  ManeuverInfo : Scope  NumInputPorts=6
      settings: TimeSpan=5  ActiveDisplayYMinimum=-0.125  ActiveDisplayYMaximum=1.125  DataLoggingMaxPoints=20000  DataLoggingDecimation=10
  ManeuverState[] : Subsystem
      mask Display: disp('')
  ManeuverTime[s] : Subsystem
      mask Display: disp('')
  MdlControl : Scope  NumInputPorts=2
      settings: TimeSpan=5  DataLoggingMaxPoints=20000  DataLoggingDecimation=10
  ModeSignals : Scope  NumInputPorts=8
      settings: TimeSpan=5  DataLoggingMaxPoints=20000  DataLoggingDecimation=10  DataLoggingVariableName=ScopeData2
  Mode_AccBr[1Stim|2Driver] : Subsystem
      mask Display: disp('')
  Mode_AdaptVeloctiyToRoad[1Off|2On] : Subsystem
      mask Display: disp('')
  Mode_GearClutch[1Stim|2Driver|3OpenClutch|4RefGear] : Subsystem
      mask Display: disp('')
  Mode_LatCtrl[1Pos|2Yaw] : Subsystem
      mask Display: disp('')
  Mode_RelativeLane[0CenterLane|1PreferredLane] : Subsystem
      mask Display: disp('')
  Mode_SelectorLever[1Stim|2Driver] : Subsystem
      mask Display: disp('')
  Mode_TrafficDriver[1Off|2On] : Subsystem
      mask Display: disp('')
  Pos_AccPedal_Maneuver[%] : Subsystem
      mask Display: disp('')
  Pos_BrakePedal_Maneuver[%] : Subsystem
      mask Display: disp('')
  Pos_ClutchPedal_Maneuver[%] : Subsystem
      mask Display: disp('')
  ReferenceVelocity : Scope  NumInputPorts=4
      settings: TimeSpan=5  DataLoggingMaxPoints=20000  DataLoggingDecimation=10  DataLoggingVariableName=ScopeData3
  Reset_VehicleStates[0|1] : Subsystem
      mask Display: disp('')
  RoadControl[] : Subsystem
      mask Display: disp('')
  SelectorLever_Maneuver[] : Subsystem
      mask Display: disp('')
  TurnLights : Scope
      settings: TimeSpan=5  DataLoggingMaxPoints=20000  DataLoggingDecimation=10  DataLoggingVariableName=ScopeData2
  d_Maneuver[m] : Subsystem
      mask Display: disp('')
  s_local[m] : Subsystem
      mask Display: disp('')
  t_local[s] : Subsystem
      mask Display: disp('')
  v_Vehicle_Ref_Maneuver[km|h] : Subsystem
      mask Display: disp('')
  v_Vehicle_Ref_Maneuver[m|s] : Subsystem
      mask Display: disp('')
  v_Vehicle_Ref_Preview_Maneuver[m|s] : Subsystem
      mask Display: disp('')
  v_Vehicle_Ref_Preview_State[0Invalid|1CurrentSeg|2NextSeg] : Subsystem
      mask Display: disp('')
  wires:
  SelectorLever_Maneuver[]/1(Out1) -> Driver/6  "SelectorLever_Maneuver[]"
  Gear_Maneuver[]/1(Out1) -> Driver/5  "Gear_Maneuver[]"
  Angle_SteeringWheel_Maneuver[deg]/1(Out1) -> Driver/4  "Angle_SteeringWheel_Maneuver[deg]"
  Pos_ClutchPedal_Maneuver[%]/1(Out1) -> Driver/3  "Pos_ClutchPedal_Maneuver[%]"
  Pos_BrakePedal_Maneuver[%]/1(Out1) -> Driver/2  "Pos_BrakePedal_Maneuver[%]"
  Pos_AccPedal_Maneuver[%]/1(Out1) -> Driver/1  "Pos_AccPedal_Maneuver[%]"
  LaneIdx_Maneuver[]/1(Out1) -> LateralOffset/2  "LaneIdx_Maneuver[]"
  d_Maneuver[m]/1(Out1) -> LateralOffset/1  "d_Maneuver[m]"
  v_Vehicle_Ref_Preview_State[0Invalid|1CurrentSeg|2NextSeg]/1(Out1) -> ReferenceVelocity/4  "v_Vehicle_Ref_Preview_State[0Invalid|1CurrentSeg|2NextSeg]"
  v_Vehicle_Ref_Preview_Maneuver[m|s]/1(Out1) -> ReferenceVelocity/3  "v_Vehicle_Ref_Preview_Maneuver[m|s]"
  v_Vehicle_Ref_Maneuver[m|s]/1(Out1) -> ReferenceVelocity/1  "v_Vehicle_Ref_Maneuver[m|s]"
  Bus Selector4/12 -> v_Vehicle_Ref_Preview_State[0Invalid|1CurrentSeg|2NextSeg]/1(In1)  "<v_Vehicle_Ref_Preview_State[0Invalid|1CurrentSeg|2NextSeg]>"
  Bus Selector4/11 -> v_Vehicle_Ref_Preview_Maneuver[m|s]/1(In1)  "<v_Vehicle_Ref_Preview_Maneuver[m|s]>"
  Bus Selector4/9 -> v_Vehicle_Ref_Maneuver[m|s]/1(In1)  "<v_Vehicle_Ref_Maneuver[m|s]>"
  Bus Selector4/8 -> LaneIdx_Maneuver[]/1(In1)  "<LaneIdx_Maneuver[]>"
  Bus Selector4/7 -> d_Maneuver[m]/1(In1)  "<d_Maneuver[m]>"
  Bus Selector4/6 -> SelectorLever_Maneuver[]/1(In1)  "<SelectorLever_Maneuver[]>"
  Bus Selector4/5 -> Gear_Maneuver[]/1(In1)  "<Gear_Maneuver[]>"
  Bus Selector4/4 -> Angle_SteeringWheel_Maneuver[deg]/1(In1)  "<Angle_SteeringWheel_Maneuver[deg]>"
  Bus Selector4/3 -> Pos_ClutchPedal_Maneuver[%]/1(In1)  "<Pos_ClutchPedal_Maneuver[%]>"
  Bus Selector4/2 -> Pos_BrakePedal_Maneuver[%]/1(In1)  "<Pos_BrakePedal_Maneuver[%]>"
  Bus Selector4/1 -> Pos_AccPedal_Maneuver[%]/1(In1)  "<Pos_AccPedal_Maneuver[%]>"
  Mode_RelativeLane[0CenterLane|1PreferredLane]/1(Out1) -> ModeSignals/8  "Mode_RelativeLane[0CenterLane|1PreferredLane]"
  Mode_TrafficDriver[1Off|2On]/1(Out1) -> ModeSignals/7  "Mode_TrafficDriver[1Off|2On]"
  Mode_SelectorLever[1Stim|2Driver]/1(Out1) -> ModeSignals/6  "Mode_SelectorLever[1Stim|2Driver]"
  Mode_AdaptVeloctiyToRoad[1Off|2On]/1(Out1) -> ModeSignals/5  "Mode_AdaptVeloctiyToRoad[1Off|2On]"
  Mode_LatCtrl[1Pos|2Yaw]/1(Out1) -> ModeSignals/4  "Mode_LatCtrl[1Pos|2Yaw]"
  LatDriver[1LatCtrl|2LatCtrl2]/1(Out1) -> ModeSignals/3  "LatDriver[1LatCtrl|2LatCtrl2]"
  Mode_GearClutch[1Stim|2Driver|3OpenClutch|4RefGear]/1(Out1) -> ModeSignals/2  "Mode_GearClutch[1Stim|2Driver|3OpenClutch|4RefGear]"
  Mode_AccBr[1Stim|2Driver]/1(Out1) -> ModeSignals/1  "Mode_AccBr[1Stim|2Driver]"
  Bus Selector3/8 -> Mode_RelativeLane[0CenterLane|1PreferredLane]/1(In1)  "<Mode_RelativeLane[0CenterLane|1PreferredLane]>"
  Bus Selector3/7 -> Mode_TrafficDriver[1Off|2On]/1(In1)  "<Mode_TrafficDriver[1Off|2On]>"
  Bus Selector3/6 -> Mode_SelectorLever[1Stim|2Driver]/1(In1)  "<Mode_SelectorLever[1Stim|2Driver]>"
  Bus Selector3/5 -> Mode_AdaptVeloctiyToRoad[1Off|2On]/1(In1)  "<Mode_AdaptVelocityToRoad[1Off|2On]>"
  Bus Selector3/4 -> Mode_LatCtrl[1Pos|2Yaw]/1(In1)  "<Mode_LatCtrl[1Pos|2Yaw]>"
  Bus Selector3/3 -> LatDriver[1LatCtrl|2LatCtrl2]/1(In1)  "<LatDriver[1LatCtrl1|2LatCtrl2]>"
  Bus Selector3/2 -> Mode_GearClutch[1Stim|2Driver|3OpenClutch|4RefGear]/1(In1)  "<Mode_GearClutch[1Stim|2Driver|3OpenClutch|4RefGear]>"
  Bus Selector3/1 -> Mode_AccBr[1Stim|2Driver]/1(In1)  "<Mode_AccBr[1Stim|2Driver]>"
  RoadControl[]/1(Out1) -> MdlControl/2  "RoadControl[]"
  Reset_VehicleStates[0|1]/1(Out1) -> MdlControl/1  "Reset_VehicleStates[0|1]"
  Bus Selector2/2 -> RoadControl[]/1(In1)  "<RoadControl[]>"
  Bus Selector2/1 -> Reset_VehicleStates[0|1]/1(In1)  "<Reset_VehicleStates[0|1]>"
  Bus Selector/4 -> Bus Selector4/1  "<RefSignals>"
  Bus Selector/3 -> Bus Selector3/1  "<ModeSignals>"
  Bus Selector/2 -> Bus Selector2/1  "<MdlControl>"
  ManeuverState[]/1(Out1) -> ManeuverInfo/6  "ManeuverState[]"
  ManeuverTime[s]/1(Out1) -> ManeuverInfo/5  "ManeuverTime[s]"
  s_local[m]/1(Out1) -> ManeuverInfo/4  "s_local[m]"
  t_local[s]/1(Out1) -> ManeuverInfo/3  "t_local[s]"
  CurrentSequence[]/1(Out1) -> ManeuverInfo/2  "CurrentSequence[]"
  CurrentSegment[]/1(Out1) -> ManeuverInfo/1  "CurrentSegment[]"
  Bus Selector1/2 -> CurrentSequence[]/1(In1)  "<CurrentSequence[]>"
  Bus Selector1/6 -> ManeuverState[]/1(In1)  "<ManeuverState[]>"
  Bus Selector1/5 -> ManeuverTime[s]/1(In1)  "<ManeuverTime[s]>"
  Bus Selector1/4 -> s_local[m]/1(In1)  "<s_local[m]>"
  Bus Selector1/3 -> t_local[s]/1(In1)  "<t_local[s]>"
  Bus Selector1/1 -> CurrentSegment[]/1(In1)  "<CurrentSegment[]>"
  Bus Selector/1 -> Bus Selector1/1  "<Info>"
  In/1 -> Bus Selector/1
  Bus Selector/5 -> Bus Selector5/1  "<UserSignals_Customized>"
  Bus Selector5/1 -> ASM_Vehicle_TurnLights[]/1(In1)  "<ASM_Vehicle_TurnLights[]>"
  ASM_Vehicle_TurnLights[]/1(Out1) -> TurnLights/1  "ASM_Vehicle_TurnLights[]"
  Bus Selector4/10 -> v_Vehicle_Ref_Maneuver[km|h]/1(In1)  "<v_Vehicle_Ref_Maneuver[km|h]>"
  v_Vehicle_Ref_Maneuver[km|h]/1(Out1) -> ReferenceVelocity/2  "v_Vehicle_Ref_Maneuver[km|h]"

== system ASM_Traffic_MultiCore/Environment/Maneuver/UserInterface/PAR_Plant ==
  note: User Interface
  note: -------------
  note: -------------
  note: -------------
  note: External Signals
  note: Plant
  note: -------------
  note: Inport colors:
  note: Control
  Interface_In : Inport
  Bus Creator2 : BusCreator  Inputs=7
  Bus Selector1 : BusSelector  OutputSignals=Interface_In
  Bus Selector3 : BusSelector  OutputSignals=ExternalModel.Sw_MasterBrakeCylinder_Mode[1linear|2physical|3Booster]
  Enable_External_Interfaces : Subsystem
      mask Display: disp('Enable External Interfaces')
  MANEUVER_SELECT_SWITCH : ASM_Environment_lib/Environment/Maneuver/MANEUVER_SELECT_SWITCH  Tag=ASM_SUBCOMPONENT  Sw_Maneuver_Select=MDL.Environment.SW_Maneuver_Select.v  ASMProperties=struct('Name','MANEUVER_SELECT_SWITCH','Version','3.0','Library','ASM_Environment_lib')  ASMInstanceName=maneuver_select_switch  ASMInstanceID=1
  ManeuverControl : Subsystem
      mask Display: disp('Maneuver Control')
  ManeuverSettings : Subsystem
      mask Display: disp('Maneuver Settings')
  ManualControl : Subsystem
      mask Display: disp('Manual Control')
  SimulationControl : Subsystem
      mask Display: disp('Simulation Control')
  Vehicle_Inits : Subsystem
      mask Display: disp('Vehicle Inits')
  Out : Outport  VectorParamsAs1DForOutWhenUnconnected=off
  wires:
  Enable_External_Interfaces/1(Out) -> Bus Creator2/7
  ManeuverSettings/1(Out1) -> Bus Creator2/3
  Vehicle_Inits/1(Out1) -> Bus Creator2/6
  MANEUVER_SELECT_SWITCH/1 -> Bus Creator2/1  "Sw_ManeuverSelect[1_6]"
  SimulationControl/1(Out1) -> Bus Creator2/4
  ManeuverControl/1(Out1) -> Bus Creator2/2
  ManualControl/1(Out1) -> Bus Creator2/5
  Bus Creator2/1 -> Out/1  "UserInterface"
  Interface_In/1 -> Bus Selector1/1
  Bus Selector3/1 -> ManeuverSettings/1(External_In)  "<Sw_MasterBrakeCylinder_Mode[1linear|2physical|3Booster]>"
  Bus Selector1/1 -> Bus Selector3/1  "<Interface_In>"

== system ASM_Traffic_MultiCore/Environment/Road/PlantModel/ASMSignalCollector ==
  SwitchRoad[0BasicRoad|1StandardRoad] : Inport
  Bus Creator : BusCreator  Inputs=13
  Bus Creator1 : BusCreator  Inputs=2
  Bus Creator2 : BusCreator  Inputs=2
  Bus Selector1 : BusSelector  OutputSignals=Road_Init,Road_ASMVeh,Road_ContactPoints,Road_Preview  OutputAsBus=on
  Bus Selector2 : BusSelector  OutputSignals=Road_Info,Road_TrafficFellows,UserSignals,TrafficObject_Data[]
  Bus Selector4 : BusSelector  OutputSignals=Road_Init,Road_ASMVeh,Road_ContactPoints,Road_Preview
  Bus to Vector : BusToVector
  Demux : Demux  Outputs=[3,3]
  Switch1 : Switch  Threshold=0.5  SaturateOnIntegerOverflow=off  InputSameDT=off
  Unit Delay : UnitDelay  SampleTime=-1
  Road_Signals : Outport  VectorParamsAs1DForOutWhenUnconnected=off
  wires:
  Bus Selector2/4 -> Bus Creator/8  "<TrafficObject_Data[]>"
  Bus Selector2/3 -> Bus Creator/7  "<UserSignals>"
  Bus Selector2/2 -> Bus Creator/6  "<Road_TrafficFellows>"
  Bus Selector2/1 -> Bus Creator/5  "<Road_Info>"
  [ASMBUS_Environment_Lane_Network] -> Bus Creator/13  "Lane_Network"
  Bus Creator1/1 -> Bus Creator/12  "LaneSensor_Dynamic"
  [ASMBUS_Environment_LaneSensor_Dynamic_Output] -> Bus Creator1/2  "Sensor_Output"
  [ASMBUS_Environment_LaneSensor_Dynamic_Parameters] -> Bus Creator1/1  "Parameters"
  [ASMBUS_Environment_Ambient] -> Bus Creator/11
  [ASMBUS_Environment_Customized_UserSignals] -> Bus Creator/9
  [ASMBUS_Environment_PosVehGPS] -> Bus Creator/10
  Bus Selector4/4 -> Bus Creator/4  "<Road_Preview>"
  Bus Selector4/3 -> Bus Creator/3  "<Road_ContactPoints>"
  Bus Selector4/2 -> Bus Creator/2  "<Road_ASMVeh>"
  [ASMBUS_Environment_StandardRoad] -> Bus Selector1/1, Bus Selector2/1
  [ASMBUS_Environment_BasicRoads] -> Switch1/3
  Bus Selector1/1 -> Switch1/1
  SwitchRoad[0BasicRoad|1StandardRoad]/1 -> Switch1/2
  Switch1/1 -> Bus Selector4/1
  Bus Creator/1 -> Road_Signals/1  "Road"
  Bus to Vector/1 -> Demux/1
  Bus Selector4/1 -> Unit Delay/1  "<Road_Init>"
  Demux/1 -> Bus Creator2/1  "Pos_Vehicle_Init_CoorSys_E[x;y;z][m]"
  Demux/2 -> Bus Creator2/2  "Angle_Vehicle_Init_CoorSys_E[x;y;z][rad]"
  Unit Delay/1 -> Bus to Vector/1
  Bus Creator2/1 -> Bus Creator/1  "Road_Init"

== system ASM_Traffic_MultiCore/Environment/Road/PlantModel/Customize_UserSignals ==
  UserSignals_In : Inport
  Bus Creator : BusCreator  Inputs=10
  Bus Selector1 : BusSelector  OutputSignals=User1[],User2[],User3[],User4[],User5[],User6[],User7[],User8[],User9[],User10[]
  CustomizedUserSignals : Subsystem
  User10 : Subsystem
      mask Display: disp('')
  User4 : Subsystem
      mask Display: disp('')
  User5 : Subsystem
      mask Display: disp('')
  User6 : Subsystem
      mask Display: disp('')
  User7 : Subsystem
      mask Display: disp('')
  User8 : Subsystem
      mask Display: disp('')
  User9 : Subsystem
      mask Display: disp('')
  ASMSignalBus : Outport  VectorParamsAs1DForOutWhenUnconnected=off
  UserSignals_Customized : Outport  Port=2  VectorParamsAs1DForOutWhenUnconnected=off
  wires:
  CustomizedUserSignals/3(Const_Offset_Long[deg]) -> Bus Creator/3
  CustomizedUserSignals/2(Const_Offset_Lat[deg]) -> Bus Creator/2
  CustomizedUserSignals/1(GPS_Method[]) -> Bus Creator/1
  Bus Selector1/3 -> CustomizedUserSignals/3(User3[])  "<User3[]>"
  Bus Selector1/2 -> CustomizedUserSignals/2(User2[])  "<User2[]>"
  Bus Selector1/1 -> CustomizedUserSignals/1(User1[])  "<User1[]>"
  Bus Creator/1 -> ASMSignalBus/1, UserSignals_Customized/1  "UserSignals_Customized"
  UserSignals_In/1 -> Bus Selector1/1
  User10/1(Out1) -> Bus Creator/10  "User10[]"
  Bus Selector1/10 -> User10/1(In1)  "<User10[]>"
  User9/1(Out2) -> Bus Creator/9  "User9[]"
  Bus Selector1/9 -> User9/1(In2)  "<User9[]>"
  User4/1(Out1) -> Bus Creator/4  "User4[]"
  Bus Selector1/4 -> User4/1(In1)  "<User4[]>"
  Bus Selector1/5 -> User5/1(In1)  "<User5[]>"
  Bus Selector1/6 -> User6/1(In1)  "<User6[]>"
  Bus Selector1/7 -> User7/1(In1)  "<User7[]>"
  Bus Selector1/8 -> User8/1(In2)  "<User8[]>"
  User8/1(Out2) -> Bus Creator/8  "User8[]"
  User7/1(Out1) -> Bus Creator/7  "User7[]"
  User6/1(Out1) -> Bus Creator/6  "User6[]"
  User5/1(Out1) -> Bus Creator/5  "User5[]"
